simulink model "follow_car"  (R2026a)
settings: Solver=VariableStepAuto  StopTime=25.0
libraries: robotmobilelib x1
settings Model: Creator=hanjiatong  LastModifiedBy=hanjiatong

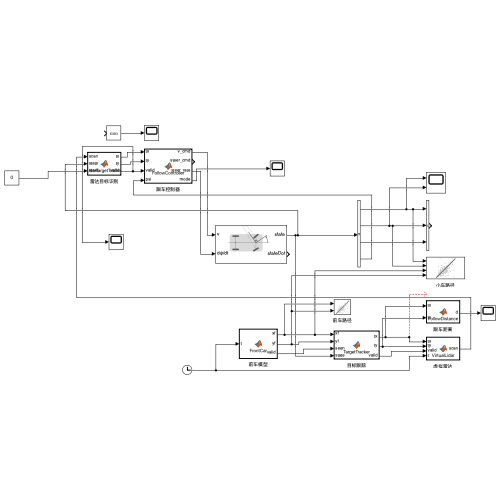
[thumbnail: Simulink's stored preview of the top-level diagram]
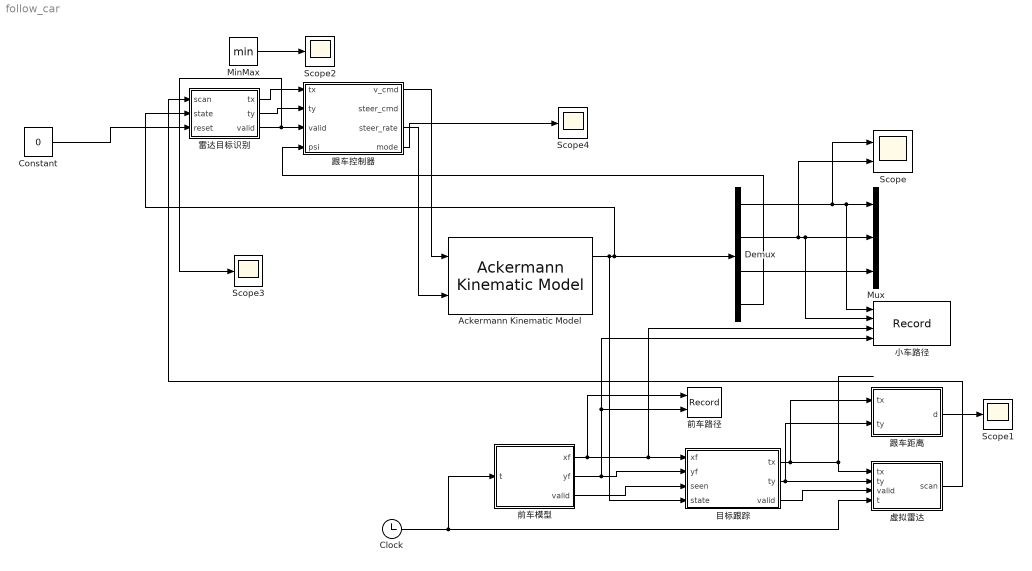
== system follow_car ==
  Ackermann Kinematic Model : robotmobilelib/Ackermann Kinematic Model  WheelBase=0.144  VehicleSpeedRange=[-inf inf]  MaxSteeringAngle=0.25  InitialState=[0;0;0;0]  SimulateUsing=Interpreted execution
  Clock : Clock
  Constant : Constant  Value=0
  Demux : Demux
      settings: DisplayOption=none
  MinMax : MinMax
  Mux : Mux  Inputs=3
  Scope : Scope  NumInputPorts=2
      settings: ActiveDisplayYMinimum=0.75000000000000011  ActiveDisplayYMaximum=3.25
  Scope{1..4} (4 alike) : Scope
      Scope1 settings: ActiveDisplayYMinimum=0.67044710971648724  ActiveDisplayYMaximum=1.1988549089933207
      Scope2 settings: ActiveDisplayYMinimum=-0.4778182824395929  ActiveDisplayYMaximum=11.164202031382176  DataLoggingVariableName=ScopeData2
      Scope3 settings: ActiveDisplayYMinimum=-0.12499999999999997  ActiveDisplayYMaximum=1.125  DataLoggingVariableName=ScopeData3
      Scope4 settings: ActiveDisplayYMinimum=-0.12499999999999997  ActiveDisplayYMaximum=1.125  DataLoggingVariableName=ScopeData4
  前车模型 : MATLAB Function  TreatAsAtomicUnit=on
  前车路径 : Record  NumPorts=2.0  FileSettingsInternal="{\"entries\":[{\"content\":{\"excelSettings\":{\"content\":{},\"type\":\"Streamout.ExcelSettings\"},\"parquetSettings\":{\"content\":{},\"type\":\"Streamout.ParquetSettings\"}},\"type\":\"Streamout.FileSettingStorage\",\"uuid\":\"\"}],\"packageUris\":[\"http:\\/\\/schema.mathworks.com\\/mf0\\/streamout_blocks\\/R2020a\"],\"version\":\"1.0\"}"  FrameSettings=[0, 0]  Layout=[1 1]  SignalsInternal="{\"entries\":[{\"content\":{\"signals\":[{\"content\":{\"blockPath\":[],\"dimensions\":[1],\"domain\":\"\",\"lineColor\":\"#a2142f\",\"plots\":[ 1 ],\"port\":1,\"sid\":[\"\"],\"signalID\":1,\"signalName\":\"前车模型:1\"},\"type\":\"RecordBlkView.Signal\",\"uuid\":\"\"},{\"content\":{\"blockPath\":[],\"dimensions\":[1],\"domain\":\"\",\"lineColor\":\"#139fff\",\"plots\":[ 1 ],\"port\":2,\"sid\":[\"\"],\"signalID\":2,\"signalName\":\"前车模型:2\"},\"type\":\"RecordBlkView.Signal\",\"uuid\":\"\"}]},\"type\":\"RecordBlkView.InputSignals\",\"uuid\":\"\"}],\"packageUris\":[\"http:\\/\\/schema.mathworks.com\\/mf0\\/streamout_blocks\\/R2020a\"],\"version\":\"1.0\"}"  VisualizationBindings="{\"xyplotplugin\":{\"info\":[{\"series\":[{\"bindingParametersList\":[{\"parameter\":\"X-Axis\",\"signalID\":1,\"signalName\":\"前车模型:1\"},{\"parameter\":\"Y-Axis\",\"signalID\":2,\"signalName\":\"前车模型:2\"}],\"seriesID\":0}],\"subplotID\":1}]}}"  CompatibilityTag=XY
  小车路径 : Record  NumPorts=4.0  FileSettingsInternal="{\"entries\":[{\"content\":{\"excelSettings\":{\"content\":{},\"type\":\"Streamout.ExcelSettings\"},\"parquetSettings\":{\"content\":{},\"type\":\"Streamout.ParquetSettings\"}},\"type\":\"Streamout.FileSettingStorage\",\"uuid\":\"\"}],\"packageUris\":[\"http:\\/\\/schema.mathworks.com\\/mf0\\/streamout_blocks\\/R2020a\"],\"version\":\"1.0\"}"  FrameSettings=[0, 0, 0, 0]  Layout=[1 1]  SignalsInternal="{\"entries\":[{\"content\":{\"signals\":[{\"content\":{\"blockPath\":[],\"dimensions\":[1],\"domain\":\"\",\"lineColor\":\"#a2142f\",\"plots\":[ 1 ],\"port\":1,\"sid\":[\"\"],\"signalID\":1,\"signalName\":\"Demux:1\"},\"type\":\"RecordBlkView.Signal\",\"uuid\":\"\"},{\"content\":{\"blockPath\":[],\"dimensions\":[1],\"domain\":\"\",\"lineColor\":\"#139fff\",\"plots\":[ 1 ],\"port\":2,\"sid\":[\"\"],\"signalID\":2,\"signalName\":\"Demux:2\"},\"type\":\"RecordBlkView.Signal\",\"uuid\":\"\"},{\"content\":{\"blockPath\":[],\"dimensions\":[1],\"domain\":\"\",\"lineColor\":\"#ff13a6\",\"lineWidth\":2,\"plots\":[ 1 ],\"port\":3,\"sid\":[\"\"],\"signalID\":3,\"signalName\":\"前车模型:1\"},\"type\":\"RecordBlkView.Signal\",\"uuid\":\"\"},{\"content\":{\"blockPath\":[],\"dimensions\":[1],\"domain\":\"\",\"lineColor\":\"#fe330a\",\"lineWidth\":2,\"plots\":[ 1 ],\"port\":4,\"sid\":[\"\"],\"signalID\":4,\"signalName\":\"前车模型:2\"},\"type\":\"RecordBlkView.Signal\",\"uuid\":\"\"}]},\"type\":\"RecordBlkView.InputSignals\",\"uuid\":\"\"}],\"packageUris\":[\"http:\\/\\/schema.mathworks.com\\/mf0\\/streamout_blocks\\/R2020a\"],\"version\":\"1.0\"}"  VisualizationBindings="{\"xyplotplugin\":{\"info\":[{\"series\":[{\"bindingParametersList\":[{\"parameter\":\"X-Axis\",\"signalID\":1,\"signalName\":\"Demux:1\"},{\"parameter\":\"Y-Axis\",\"signalID\":2,\"signalName\":\"Demux:2\"}],\"seriesID\":0},{\"bindingParametersList\":[{\"parameter\":\"X-Axis\",\"signalID\":3,\"signalName\":\"前车模型:1\"},{\"parameter\":\"Y-Axis\",\"signalID\":4,\"signalName\":\"前车模型:2\"}],\"seriesID\":1}],\"subplotID\":1}]}}"  CompatibilityTag=XY
  目标跟踪 : MATLAB Function  TreatAsAtomicUnit=on
  虚拟雷达 : MATLAB Function  TreatAsAtomicUnit=on
  跟车控制器 : MATLAB Function  TreatAsAtomicUnit=on
  跟车距离 : MATLAB Function  TreatAsAtomicUnit=on
  雷达目标识别 : MATLAB Function  TreatAsAtomicUnit=on
  wires:
  跟车距离/1(d) -> Scope1/1
  目标跟踪/2(ty) -> 跟车距离/2(ty), 虚拟雷达/2(ty)
  Demux/2 -> 小车路径/2, Mux/2, Scope/2
  Demux/1 -> Mux/1, 小车路径/1, Scope/1
  前车模型/3(valid) -> 目标跟踪/3(seen)
  前车模型/1(xf) -> 目标跟踪/1(xf), 小车路径/3, 前车路径/1
  目标跟踪/1(tx) -> 虚拟雷达/1(tx), 跟车距离/1(tx)
  Demux/3 -> Mux/3
  Ackermann Kinematic Model/1 -> 目标跟踪/4(state), 雷达目标识别/2(state), Demux/1
  虚拟雷达/1(scan) -> 雷达目标识别/1(scan)
  目标跟踪/3(valid) -> 虚拟雷达/3(valid)
  前车模型/2(yf) -> 前车路径/2, 小车路径/4, 目标跟踪/2(yf)
  Clock/1 -> 前车模型/1(t), 虚拟雷达/4(t)
  雷达目标识别/2(ty) -> 跟车控制器/2(ty)
  跟车控制器/3(steer_rate) -> Ackermann Kinematic Model/2
  跟车控制器/1(v_cmd) -> Ackermann Kinematic Model/1
  雷达目标识别/3(valid) -> Scope3/1, 跟车控制器/3(valid)
  雷达目标识别/1(tx) -> 跟车控制器/1(tx)
  Demux/4 -> 跟车控制器/4(psi)
  MinMax/1 -> Scope2/1
  Constant/1 -> 雷达目标识别/3(reset)
  跟车控制器/4(mode) -> Scope4/1

== matlab function follow_car/跟车控制器 ==
  settings: updateMethod=DISCRETE  sampleTime=0.02
  data: tx input; v_cmd output; ty input; valid input; psi input; steer_cmd output; steer_rate output; mode output

function [v_cmd, steer_cmd, steer_rate, mode] = ...
    FollowController(tx, ty, valid, psi)
%#codegen

% 自动跟车控制器
% tx, ty：前车相对位置
% valid：目标是否有效
% psi：当前转向角

% ===== 1. 状态变量初始化 =====

persistent v_last steer_last d_last d_rate_f e_int

if isempty(v_last)
    v_last = 0;
    steer_last = 0;
    d_last = -1;
    d_rate_f = 0;
    e_int = 0;
end

Ts = 0.02;
L = 0.144;

% ===== 2. 计算跟车距离 =====

d = hypot(tx, ty);
d_ref = 0.7;

% ===== 3. 安全停车判断 =====

if ~valid || ~isfinite(d) || ...
   tx <= 0 || d < 0.5 || d > 2.0

    v_cmd = 0;
    steer_cmd = 0;
    steer_rate = 0;
    mode = 0;

    if valid && d < 0.5
        mode = 2;
    end

    v_last = 0;
    steer_last = 0;
    d_last = -1;
    d_rate_f = 0;
    e_int = 0;
    return;
end

% ===== 4. 相对速度估计 =====

if d_last < 0
    d_rate_f = 0;
else
    d_rate = (d - d_last) / Ts;

    % 限制异常变化
    d_rate = max(-1, min(1, d_rate));

    % 一阶低通滤波
    alpha = 0.2;
    d_rate_f = (1-alpha)*d_rate_f ...
             + alpha*d_rate;
end

d_last = d;

% ===== 5. PI + 相对速度反馈 =====

Kp = 0.8;
Ki = 0.25;
Kd = 1.0;

e = d - d_ref;

% 积分误差
e_int = e_int + e*Ts;
e_int = max(-0.5, min(0.6, e_int));

% 距离控制 + 相对速度反馈
v_target = Kp*e + Ki*e_int + Kd*d_rate_f;

% 速度限制
v_target = max(0, min(0.25, v_target));

% ===== 预测制动 =====

% 两车接近速度
v_close = max(0, -d_rate_f);

% 假设最大制动减速度
a_brake = 0.5;

% 估算制动距离，考虑0.1秒响应延迟
d_brake = v_close^2/(2*a_brake) ...
    + v_close*0.1;

% 提前制动：接近目标车距时
if v_close > 0.05 && ...
        d <= d_ref + d_brake + 0.03

    v_target = 0;
    e_int = 0;
end

% 已经达到或小于目标距离，禁止继续前进
if d <= d_ref
    v_target = 0;
    e_int = 0;
end

% ===== 6. 加减速限制 =====

dv = v_target - v_last;

dv = max(-0.5*Ts, min(0.3*Ts, dv));

v_cmd = v_last + dv;
v_last = v_cmd;

% ===== 7. 转向控制 =====

steer_target = atan2(2*L*ty, max(d,0.25)^2);

% 转向角限制
steer_target = max(-0.49, ...
                   min(0.32, steer_target));

% 转向速率限制
ds = steer_target - steer_last;

ds = max(-0.8*Ts, min(0.8*Ts, ds));

steer_cmd = steer_last + ds;
steer_last = steer_cmd;

% Ackermann 转向角速度
steer_rate = (steer_cmd - psi) / Ts;

steer_rate = max(-0.8, min(0.8, steer_rate));

mode = 1;

end

== matlab function follow_car/前车模型 ==
  data: t input; xf output; yf output; valid output

function [xf, yf, valid] = FrontCar(t)
%#codegen

% 前车速度
v = 0.16;

% 转弯半径
R = 1.5;

% 初始位置
x0 = 1.2;

% 0~6秒：直行
if t <= 6
    xf = x0 + v*t;
    yf = 0;

% 6~12秒：向左转弯
elseif t <= 12
    a = v/R*(t-6);
    xf = x0 + 6*v + R*sin(a);
    yf = R*(1-cos(a));

% 12~18秒：继续直行
else
    a = v/R*6;
    dt = min(t-12, 6);

    xf = x0 + 6*v + R*sin(a) + v*dt*cos(a);
    yf = R*(1-cos(a)) + v*dt*sin(a);
end

% 21秒时模拟目标丢失
valid = (t < 21);
end

== matlab function follow_car/目标跟踪 ==
  data: xf input; tx output; yf input; seen input; state input; ty output; valid output

function [tx, ty, valid] = TargetTracker(xf, yf, seen, state)
%#codegen

% 后车状态
x = state(1);
y = state(2);
theta = state(3);

% 前车相对于后车的位置
dx = xf - x;
dy = yf - y;

% 转换到后车自身的坐标系
tx = cos(theta)*dx + sin(theta)*dy;
ty = -sin(theta)*dx + cos(theta)*dy;

% 跟踪信号是否有效
valid = seen && isfinite(tx) && isfinite(ty);

end

== matlab function follow_car/跟车距离 ==
  data: tx input; d output; ty input

function d = FollowDistance(tx, ty)
% 计算两车之间的距离
d = hypot(tx, ty);
end

== matlab function follow_car/虚拟雷达 ==
  data: tx input; scan output; ty input; valid input; t input

function scan = VirtualLidar(tx, ty, valid, t)
%#codegen

% 模拟720点激光雷达
scan = 10 * ones(720,1);

% 真实跟踪目标
d1 = hypot(tx,ty);
a1 = atan2(ty,tx);
w1 = atan2(0.1,max(d1,0.1));

% 干扰车辆的位置（后车坐标系）
x2 = 0.5;
y2 = -0.3;

d2 = hypot(x2,y2);
a2 = atan2(y2,x2);
w2 = atan2(0.07,d2);

% 12~16秒出现干扰车辆
interference = (t >= 12 && t < 16);

for i = 1:720

    angle = (i-1)*pi/360;

    if angle >= pi
        angle = angle - 2*pi;
    end

    % 第一辆车的雷达回波
    if valid && isfinite(tx) && isfinite(ty)

        diff1 = atan2( ...
            sin(angle-a1), cos(angle-a1));

        if abs(diff1) <= w1
            noise = 0.01*sin(0.37*i + 2*t);
            scan(i) = max(0.05,d1-0.1+noise);
        end
    end

    % 第二辆车的干扰回波
    if interference

        diff2 = atan2( ...
            sin(angle-a2), cos(angle-a2));

        if abs(diff2) <= w2
            noise2 = 0.01*sin(0.51*i + t);
            r2 = max(0.05,d2-0.07+noise2);

            % 雷达只测到射线上较近的物体
            scan(i) = min(scan(i),r2);
        end
    end

end

end

== matlab function follow_car/雷达目标识别 ==
  settings: updateMethod=DISCRETE  sampleTime=0.02
  data: scan input; tx output; ty output; valid output; state input; reset input

function [tx, ty, valid] = LidarTargetTracker(scan, state, reset)
%#codegen
% 雷达目标锁定 + 运动预测 + 数据关联
% scan: 720点雷达扫描，单位m
% state: 后车状态 [x;y;theta;psi]
% reset: 手动重新选择目标的复位信号

persistent px py vx vy locked missed

if isempty(locked)
    px = 0;
    py = 0;
    vx = 0;
    vy = 0;
    locked = false;
    missed = 0;
end

Ts = 0.02;

tx = 0;
ty = 0;
valid = false;

% 手动复位跟踪状态
if reset > 0.5
    locked = false;
    missed = 0;
    px = 0;
    py = 0;
    vx = 0;
    vy = 0;
end

% 当前后车位姿
ex = state(1);
ey = state(2);
theta = state(3);

ct = cos(theta);
st = sin(theta);

% 预测已锁定目标的世界坐标
dt = (missed + 1)*Ts;
predX = px + vx*dt;
predY = py + vy*dt;

% 当前最佳候选
bestScore = inf;
bestX = 0;
bestY = 0;
found = false;

% 点云聚类
n = 0;
sx = 0;
sy = 0;
prevR = 0;

for k = 1:721

    hit = false;
    r = 0;
    angle = 0;

    if k <= 720
        i = mod(k+359,720)+1;

        angle = (i-1)*pi/360;

        if angle >= pi
            angle = angle-2*pi;
        end

        r = scan(i);

        if isfinite(r) && ...
           r >= 0.12 && r <= 2.4 && ...
           abs(angle) <= pi/3

            hit = true;
        end
    end

    % 距离跳变说明可能进入另一个物体
    split = ~hit;

    if hit && n > 0
        if abs(r-prevR) > 0.18
            split = true;
        end
    end

    % 完成一个点云簇
    if split && n >= 3

        cx = sx/n;
        cy = sy/n;

        % 转换到世界坐标系
        wx = ex + ct*cx - st*cy;
        wy = ey + st*cx + ct*cy;

        if locked
            % 和预测位置进行匹配
            score = hypot(wx-predX, wy-predY);

            % 丢失越久，允许误差略增大
            gate = 0.18 + 0.015*min(missed,10);

            % 超过15帧不再自动重新锁定
            accept = missed < 15 && score < gate;

        else
            % 首次寻找正前方的目标
            bearing = atan2(cy,cx);

            score = hypot(cx,cy) ...
                  + 0.5*abs(bearing);

            accept = cx > 0.5 && ...
                     abs(bearing) < pi/6;
        end

        if accept && score < bestScore
            bestScore = score;
            bestX = wx;
            bestY = wy;
            found = true;
        end
    end

    if split
        n = 0;
        sx = 0;
        sy = 0;
    end

    if hit
        sx = sx + r*cos(angle);
        sy = sy + r*sin(angle);
        n = n+1;
        prevR = r;
    end
end

% 更新目标状态
if found

    if locked
        % 估算目标世界坐标系速度
        mx = (bestX-px)/dt;
        my = (bestY-py)/dt;

        % 限制异常估计
        mx = max(-0.5,min(0.5,mx));
        my = max(-0.5,min(0.5,my));

        % 平滑速度估计
        vx = 0.8*vx + 0.2*mx;
        vy = 0.8*vy + 0.2*my;
    else
        vx = 0;
        vy = 0;
    end

    px = bestX;
    py = bestY;

    locked = true;
    missed = 0;

    % 转回车体坐标系
    dx = px-ex;
    dy = py-ey;

    tx = ct*dx + st*dy;
    ty = -st*dx + ct*dy;

    valid = true;

else
    % 暂时保留跟踪记忆，但不输出有效目标
    if locked
        missed = min(missed+1,15);
    end

    valid = false;
end

end
